simulink model "pwtsimplificado"  (R2025a)
settings: Solver=ode3  StartTime=0.0  StopTime=34  FixedStep=Amostragem/10  RelTol=1e-3
InitFcn:
  | % Suprime os warnings de limite do MFeval. Eles disparam A CADA PASSO quando o pneu
  | % opera fora da faixa do .tir (frenagem forte, baixa velocidade, Fz baixo) e chegam a
  | % custar 10x o tempo de simulacao. Os valores ja sao saturados internamente pelo solver.
  | warning('off','Solver:Limits:Exceeded');
  | warning('off','Solver:CoeffChecks:Ex');
model workspace (MATLAB code in the model file):
  Bi = 250
  Bv = 168
  Pnom = 11000
  T_max = 94
  Poles = 2
  Rs = 0.0165
  Rr = 0.01858
  Lls = 7.4763e-5    (= 7.4763e-05)
  Llr = 7.4763e-5    (= 7.4763e-05)
  Lm = 1.0357e-3    (= 0.0010357)
  Ls = Lls + Lm    (= 0.001110463)
  Lr = Lm + Llr    (= 0.001110463)
  Im = 0.0071
  motor_eff = 0.874
  mc_eff = 0.95
  sigma = 1 - (Lm^2)/(Ls*Lr)    (= 0.130119156075)
  Tau_r = Lr/Rr    (= 0.0597665769645)
  Kt = (3/2)*Poles*(Lm^2/Lr)    (= 0.00289791147476)
  Req = Rs + Rr*((Lm/Lr)^2)    (= 0.0326623860801)
  Imag = 105
  Idref = Imag    (= 105)
  I_max_motor = 242*sqrt(2)
  I_max_inv = 257*sqrt(2)
  I_max = min(I_max_motor, I_max_inv)
  Amostragem = 1.25e-4    (= 0.000125)
  Modulation_Target = 0.95
  Vmax = (Bv*Modulation_Target)/sqrt(3)
  c_comp = 1.5
  wc = 2*pi*200    (= 1256.63706144)
  Kp = sigma*Ls*wc    (= 0.181574641171)
  Ki = Req*wc    (= 41.0447648632)
  Kaw = Ki/Kp    (= 226.048993398)
  wc_fw = 2*pi*15    (= 94.2477796077)
  Fw_margin = 0.95
  V_ref_fw = Vmax*Fw_margin
  We_base = 2*pi*103    (= 647.168086639)
  Kv_fw = We_base*Ls    (= 0.718656214994)
  Kp_fw = (1/Kv_fw)/3    (= 0.46382863792)
  Ki_fw = Kp_fw*(wc_fw/3)    (= 14.5716064141)
  Kaw_fw = Ki_fw/Kp_fw    (= 31.4159265359)
  Id_min_pu = 0.15
  dImag_max = 0
  dImag_min = -(1-Id_min_pu)*Imag    (= -89.25)
  f_lp_vmag = 50
  a_vmag = exp(-2*pi*f_lp_vmag*Amostragem)
  gear_ratio = 4.45
  trans_eff = 0.89
  Rw = 0.2605
  Iw = 1.20    (= 1.2)
  m = 366
  g = 9.81
  air_density = 1.225
  Af = 1.17
  Cd = 1.06
  Cr = 0.02
  L_wb = 1.56
  dist_cg_f = 0.804
  frac_rear = dist_cg_f/L_wb    (= 0.515384615385)
  h_cg = 0.295
  Fz_rear_static = m*g*frac_rear/2    (= 925.233923077)
  ClA_total = 2.11
  downforce_rear_share = 0.48
  K_transf = (m*h_cg/L_wb)/2    (= 34.6057692308)
  K_downf = 0.5*air_density*ClA_total*downforce_rear_share/2    (= 0.31017)
  b_cg_r = L_wb - dist_cg_f    (= 0.756)
  Iz = 120
  Fz_front_static = m*g*(1-frac_rear)/2    (= 869.996076923)
  downforce_front_share = 1 - downforce_rear_share    (= 0.52)
  K_downf_f = 0.5*air_density*ClA_total*downforce_front_share/2    (= 0.3360175)
  T_brake_max = 1700
  brake_bias_f = 0.70    (= 0.7)
  brake_cut = 0.15
  accel_deadzone = 2
  T_regen_max = 94
  regen_coast = 0.35
  Bi_regen = 60
  v_regen_off = 1.4
  v_regen_full = 4.0    (= 4)
  w_motor_min = 20
  regen_margin = 0.95
  regen_rate = 200
  roll_grad = 0.7
  pitch_grad = 0.5
  delta_amp = 0.03
  steer_t0 = 6.5
  steer_t1 = 9.0    (= 9)
  steer_freq = 0.5
  R_turn = 9.125
  steer_ramp = 1.0    (= 1)
  delta_max = 0.35
  steer_rate_max = 3.0    (= 3)
  delta_input = timeseries([0;0],[0;1000])
  Ca_c1 = 36392
  Ca_c2 = 1474
  mu_a = 2.6537
  mu_b = -2.225e-4    (= -0.0002225)
  Cf_shape = 1.3
  Vx_min_tire = 1.0    (= 1)
  mu_scale = 1.0    (= 1)
  Iw_f = 0.9
  Velocity = 0.1
  Wheel_Speed = 1
  Iqref = 0.1
  Vd = 0.1
  Vq = 0.1
  tirNome = 'Avon_9760_Round_2.tir'
  tirFile = ''
  tirParams = mfeval.readTIR(tirFile)
  Iq35 = 35/(Kt*Imag)    (= 115.025367833)
  Iq94 = 94/(Kt*Imag)    (= 308.92527361)
  K_us_est = (m*g*(1-frac_rear))/(2*Ca_c1*sin(2*atan(Fz_front_static/Ca_c2)))           - (m*g*frac_rear)/(2*Ca_c1*sin(2*atan(Fz_rear_static/Ca_c2)))
  pistaArq = fullfile(raizModelo,'data','pista_amp226.mat')
  pista_ = load(pistaArq)
  pista_ = pista_.pista
  trk_passo = 0.5
  s_ = transpose(0 : trk_passo : pista_.Lap - trk_passo)
  trk_x = interp1(pista_.s, pista_.x,     s_)
  trk_y = interp1(pista_.s, pista_.y,     s_)
  trk_k = interp1(pista_.s, pista_.kappa, s_)
  trk_passo = 0.5
  trk_x = [0;1]
  trk_y = [0;0]
  trk_k = [0;0]
  pp_Ld_min = 4.0    (= 4)
  pp_Ld_k = 0.55
  pp_v_max = 22.0    (= 22)
  pp_ay_max = 9.0    (= 9)
  pp_kp_v = 0.35
  pp_kp_b = 0.30    (= 0.3)
  pp_v_banda = 0.8
  pp_frn_max = 0.90    (= 0.9)
  pp_prev = 12.0    (= 12)
  pp_Ts = 0.01
  pp_ped_max = 100
  piloto_on = 1
  steer_mode = 5
  other statements: assert(Kaw_fw*Amostragem < 0.1, 'Kaw_fw alto demais'); try, raizModelo = fileparts(get_param('pwtsimplificado','FileName')); catch, raizModelo = pwd; end; for c = {fullfile(raizModelo,'data',tirNome), fullfile(raizModelo,tirNome), which(tirNome)}; if ~isempty(c{1}) && isfile(c{1}), tirFile = c{1}; break, end; end; assert(~isempty(tirFile), 'Arquivo %s nao encontrado em %s/data nem no path do MATLAB.', tirNome, raizModelo);; fprintf('--- Verificacoes ---\n');; fprintf('Kaw*Ts   = %.4f | wc*Ts = %.4f  (ambos << 1)\n', Kaw*Amostragem, wc*Amostragem);; fprintf('sigma    = %.4f (esperado 0.130) | Tau_r = %.1f ms (esperado 59.8 - se der ~35, Rr esta ERRADO)\n', sigma, Tau_; fprintf('Kt = %.4g (esperado 2.898e-3) | Req = %.4g\n', Kt, Req);; fprintf('Kp = %.3f V/A | Ki = %.1f V/(A*s) | Kaw = %.1f 1/s\n', Kp, Ki, Kaw);; fprintf('FW: Kp_fw = %.3f | Ki_fw = %.2f | Kaw_fw = %.2f | dImag_min = %.2f\n', Kp_fw, Ki_fw, Kaw_fw, dImag_min); ... (+18)
undefined symbols (not defined in the file): DiscIntNeverNeededParam, dspblkCoreblockFVToolHelper, gcbh, sigbuilder_block, Vq_lim
libraries: mcbeeMathTransformLib x4, spsControlledVoltageSourceLib x3, spsGroundLib x3, simulink x2, spsAsynchronousMachineSIUnitsLib x1, spspowerguiLib x1, mfeval_LIB x1
(part 2 of 2)

== matlab function pwtsimplificado/Pneu Dianteiro/Eixo Dianteiro ==
  data: Vx input; Fx_body output; Vy input; psi_dot input; delta input; brake input; ax_f input; Fy_body output; Fz_w output; alpha_f output; Vx_min_tire parameter double size=1; Fz_front_static parameter double size=1; K_transf parameter double size=1; K_downf_f parameter double size=1; dist_cg_f parameter double size=1; mu_scale parameter double size=1; mu_a parameter double size=1; mu_b parameter double size=1; Ca_c1 parameter double size=1; Ca_c2 parameter double size=1; Cf_shape parameter double size=1; T_brake_max parameter double size=1; brake_bias_f parameter double size=1; Rw parameter double size=1
function [Fx_body, Fy_body, Fz_w, alpha_f] = fcn(Vx, Vy, psi_dot, delta, brake, ax_f, Vx_min_tire, Fz_front_static, K_transf, K_downf_f, dist_cg_f, mu_scale, mu_a, mu_b, Ca_c1, Ca_c2, Cf_shape, T_brake_max, brake_bias_f, Rw)
%#codegen
% Eixo DIANTEIRO analitico (par de rodas), calibrado no Avon 9760 via mfeval.
% Substitui um 2o bloco MFeval, que custava ~50x o resto do modelo (roda livre
% em baixa velocidade faz o solver de transientes nao-lineares iterar demais).

Vxs = max(Vx, Vx_min_tire);

% --- carga vertical por roda: estatica - transferencia + downforce ---
Fz_w = Fz_front_static - K_transf*ax_f + K_downf_f*Vxs^2;
Fz_w = max(Fz_w, 50);

% --- angulo de deriva do eixo dianteiro ---
alpha_f = delta - atan((Vy + dist_cg_f*psi_dot)/Vxs);

% --- Magic Formula simplificada (por roda) ---
mu = mu_scale*(mu_a + mu_b*Fz_w);
D  = mu*Fz_w;
Ca = Ca_c1*sin(2*atan(Fz_w/Ca_c2));
B  = Ca/(Cf_shape*D);

% --- frenagem: forca longitudinal por roda, limitada pelo atrito ---
Fx_dem = brake*T_brake_max*brake_bias_f/2/Rw;
Fx_w   = -min(Fx_dem, D)*tanh(Vx);

% --- elipse de atrito: o que sobra vai para o lateral ---
res  = max(1 - (Fx_w/D)^2, 0);
Fy_w = sqrt(res)*D*sin(Cf_shape*atan(B*alpha_f));

% --- par de rodas + rotacao para o referencial do carro ---
Fx2 = 2*Fx_w;  Fy2 = 2*Fy_w;
Fx_body = Fx2*cos(delta) - Fy2*sin(delta);
Fy_body = Fx2*sin(delta) + Fy2*cos(delta);

== matlab function pwtsimplificado/Monitor DC/Potencia DC ==
  data: Vd input; P_dc output; Vq input; Idm input; Iqm input; I_dc output; P_recup output; mc_eff parameter double size=1; Bv parameter double size=1
function [P_dc, I_dc, P_recup] = fcn(Vd, Vq, Idm, Iqm, mc_eff, Bv)
%#codegen
% Potencia eletrica no estator. Correntes em PICO de fase -> fator 3/2.
P_ac = 1.5*(Vd*Idm + Vq*Iqm);

% As perdas do inversor sempre penalizam quem RECEBE:
%   tracao -> a bateria entrega MAIS do que o estator consome
%   regen  -> a bateria recebe MENOS do que o estator devolve
if P_ac >= 0
    P_dc = P_ac/mc_eff;
else
    P_dc = P_ac*mc_eff;
end

I_dc    = P_dc/Bv;          % negativa = carregando o acumulador
P_recup = min(P_dc, 0);     % so a parte recuperada, para integrar a energia
